simulink model "BasePerTracing_2023a"  (R2023a)
settings: Solver=FixedStepDiscrete  StartTime=0.0  StopTime=Inf  RelTol=1e-3  EnableMultiTasking=on
InitFcn:
  | mcb_pmsm_foc_qep_f28379d_data;
values from neighbouring files (symbols this model uses):
  ADCCount = ADCResolution-1    (= 4095)    [parameters.m]
  GainVsense = 4.99/(62+4.99)    (= 0.0744887296611)    [parameters.m]
  J = Jdc + Jbl    (= 7.32e-05)    [parameters.m]
  Km = 0.11    [parameters.m]
  Kpi = L/taui    (= 4.1)    [parameters.m]
  Kpv = J/(tauv*Km)    (= 0.0665454545455)    [parameters.m]
  OffsetADCINC4 = 2296    [parameters.m]
  PulseNumber = 2048*4    (= 8192)    [parameters.m]
  RadiantsPerCount = 2*pi/(PulseNumber-1)    (= 0.00076708403213)    [parameters.m]
  TaoFilterOffsetCurrent = 1    [parameters.m]
  TaoFilterOmega = 0.002    [parameters.m]
  Tii = L/R    (= 0.00128125)    [parameters.m]
  Tiv = Taom    (= 0.085)    [parameters.m]
  TSample = 0.0001    [parameters.m]
  VrefADC = 3    [parameters.m]
undefined symbols (not defined in the file or in its folder): dataType, Down, GPTRIP1SEL, GPTRIP2SEL, TZ1, TZ2, Up
libraries: c2802xlib x9, simulink x6, c280xlib x4, c2837xDlib x3, c2000lib x1, svdutilitieslib x1
(part 1 of 2)
settings Model: ExtModeTrigDuration=8  Creator=The MathWorks, Inc.  LastModifiedBy=student
settings SolverCC: AlgebraicLoopSolver=TrustRegion
settings OptimizationCC: DefaultParameterBehavior=Inlined  DefaultUnderspecifiedDataType=single  OptimizeBlockIOStorage=off  EnhancedBackFolding=on  InitFltsAndDblsToZero=on  NoFixptDivByZeroProtection=on  EfficientFloat2IntCast=on  EfficientMapNaN2IntZero=off  MaxStackSize=1024  OptimizeBlockOrder=speed  DifferentSizesBufferReuse=on  DenormalBehavior=FlushToZero  EfficientTunableParamExpr=on
settings DebuggingCC: MultiTaskDSMMsg=none  ParameterPrecisionLossMsg=none  ParameterTunabilityLossMsg=error  UnconnectedInputMsg=warning  UnconnectedOutputMsg=warning  UnconnectedLineMsg=warning
settings HardwareCC: ProdBitPerChar=16  ProdBitPerInt=16  ProdBitPerPointer=32  ProdBitPerSizeT=32  ProdBitPerPtrDiffT=32  ProdLargestAtomicInteger=Integer  ProdLargestAtomicFloat=None  ProdWordSize=16  ProdLongLongMode=on  ProdHWDeviceType=Texas Instruments->C2000
settings ModelReferenceCC: EnableRefExpFcnMdlSchedulingChecks=on
settings SFSimCC: MATLABDynamicMemAlloc=off
settings RTWCC: Description=Embedded Coder  SystemTargetFile=ert.tlc  HardwareBoard=TI Delfino F28379D LaunchPad  TemplateMakefile=ert_default_tmf  GenerateReport=on  Toolchain=Texas Instruments Code Composer Studio (C2000)  DLArmComputeVersion=19.05
settings CodeAppCC: IgnoreCustomStorageClasses=off  StateflowObjectComments=on
settings ERTTargetCC: CodeReplacementLibrary=TI C28x  ExtModeStaticAllocSize=10000  ConvertIfToSwitch=off  SuppressUnreachableDefaultCases=off  MemSecPackage=tic2000demospkg

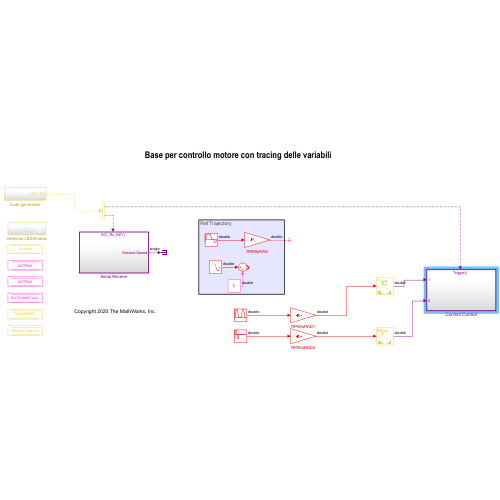
[thumbnail: Simulink's stored preview of the top-level diagram]
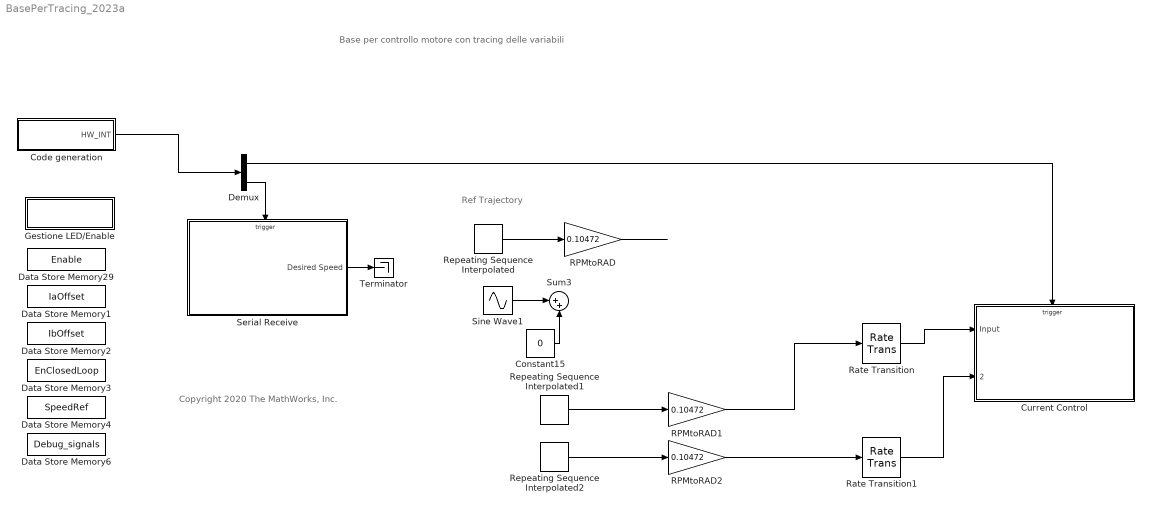
== system BasePerTracing_2023a ==
  note: Ref Trajectory
  note: Copyright 2020 The MathWorks, Inc.
  note: Base per controllo motore con tracing delle variabili
  Code generation : Subsystem
  Constant15 : Constant  Value=0
  Current Control : Subsystem
      settings: RTWSystemCode=Nonreusable function
  Data Store Memory1 : DataStoreMemory  DataStoreName=IaOffset  ReadBeforeWriteMsg=warning  WriteAfterWriteMsg=warning  WriteAfterReadMsg=warning  InitialValue=inverter.CtSensAOffset  ShowAdditionalParam=off
  Data Store Memory2 : DataStoreMemory  DataStoreName=IbOffset  ReadBeforeWriteMsg=warning  WriteAfterWriteMsg=warning  WriteAfterReadMsg=warning  InitialValue=inverter.CtSensBOffset  ShowAdditionalParam=off
  Data Store Memory29 : DataStoreMemory  DataStoreName=Enable  ReadBeforeWriteMsg=warning  WriteAfterWriteMsg=warning  WriteAfterReadMsg=warning  ShowAdditionalParam=off  OutDataTypeStr=boolean
  Data Store Memory3 : DataStoreMemory  DataStoreName=EnClosedLoop  ReadBeforeWriteMsg=warning  WriteAfterWriteMsg=warning  WriteAfterReadMsg=warning  ShowAdditionalParam=off  OutDataTypeStr=boolean
  Data Store Memory4 : DataStoreMemory  DataStoreName=SpeedRef  ShowAdditionalParam=off
  Data Store Memory6 : DataStoreMemory  DataStoreName=Debug_signals  ReadBeforeWriteMsg=warning  WriteAfterWriteMsg=warning  WriteAfterReadMsg=warning  InitialValue=5  ShowAdditionalParam=off  OutDataTypeStr=uint16
  Demux : Demux  Outputs=2
  Gestione LED/Enable : Subsystem
  RPMtoRAD : Gain  Gain=0.10472
  RPMtoRAD1 : Gain  Gain=0.10472
  RPMtoRAD2 : Gain  Gain=0.10472
  Rate Transition : RateTransition  Deterministic=off
  Rate Transition1 : RateTransition  Deterministic=off
  Repeating Sequence Interpolated : simulink/Sources/Repeating Sequence Interpolated  OutValues=[0 800 1000 1000 500 0 0 -500 -500 0].'  TimeValues=[0 0.3 0.5 1 1.2 1.4 1.7 2 2.2 2.5].'  LookUpMeth=Interpolation-Use End Values  tsamp=0.0001  OutMin=[]  OutMax=[]  OutDataTypeStr=double  OutputDataTypeScalingMode=double  OutDataType=fixdt(0,8)  OutScaling=2^-10
  Repeating Sequence Interpolated1 : simulink/Sources/Repeating Sequence Interpolated  OutValues="[0 700 700 0 0 710 710 0 0  ].'"  TimeValues=[0 0.055 0.1 0.15 0.25 0.305 0.35 0.40 0.45 ].'  LookUpMeth=Interpolation-Use End Values  tsamp=0.0001  OutMin=[]  OutMax=[]  OutDataTypeStr=double  OutputDataTypeScalingMode=double  OutDataType=fixdt(0,8)  OutScaling=2^-10
  Repeating Sequence Interpolated2 : simulink/Sources/Repeating Sequence Interpolated  OutValues=[0 12727 12727 0 0 -12727 -12727 0 0 0 0 0 0 ].'  TimeValues=[0 0.0001 0.055 0.0551 0.1 0.101 0.15 0.1501 0.25 0.305 0.35 0.40 0.45 ].'  LookUpMeth=Interpolation-Use End Values  tsamp=0.0001  OutMin=[]  OutMax=[]  OutDataTypeStr=double  OutputDataTypeScalingMode=double  OutDataType=fixdt(0,8)  OutScaling=2^-10
  Serial Receive : Subsystem  SystemSampleTime=1e-3
  Sine Wave1 : Sin  Amplitude=500  Frequency=15  SampleTime=0.0001
  Sum3 : Sum  Inputs=|++
  Terminator : Terminator
  wires:
  Code generation/1(HW_INT) -> Demux/1
  Demux/1 -> Current Control/Trigger
  Demux/2 -> Serial Receive/Trigger
  Serial Receive/1(Desired Speed) -> Terminator/1
  Rate Transition/1 -> Current Control/1(Input)
  Constant15/1 -> Sum3/2
  Repeating Sequence Interpolated/1 -> RPMtoRAD/1
  Sine Wave1/1 -> Sum3/1
  RPMtoRAD/1 -> ?
  Repeating Sequence Interpolated1/1 -> RPMtoRAD1/1
  RPMtoRAD1/1 -> Rate Transition/1
  Repeating Sequence Interpolated2/1 -> RPMtoRAD2/1
  RPMtoRAD2/1 -> Rate Transition1/1
  Rate Transition1/1 -> Current Control/2(2)

== system BasePerTracing_2023a/Code generation ==
  C28x Hardware Interrupt : c2000lib/Scheduling/C28x Hardware Interrupt  irqnumbers=[1 9]  pienumbers=[1 1]  irqpriorities=[30 50]  irqpreempts=[1 0]  showinput=off  dspchiptype=C280X
  HW_INT : Outport
  wires:
  C28x Hardware Interrupt/1 -> HW_INT/1

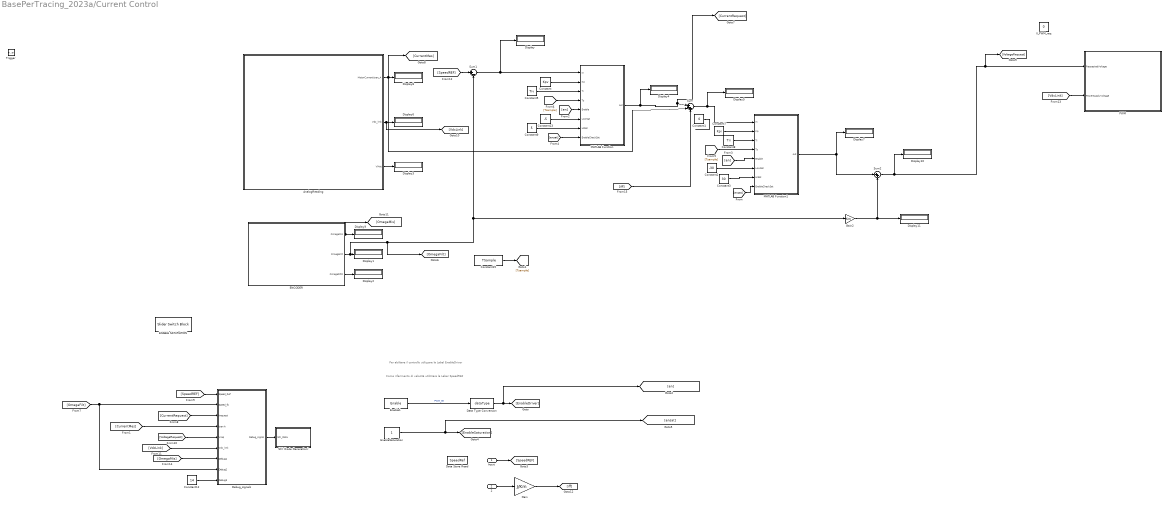
== system BasePerTracing_2023a/Current Control ==
  note: Per abilitare il controllo utilizzare la Label EnableDriver
  note: Come riferimento di velocità utilizzare la Laber SpeedREF
  Input : Inport
  2 : Inport  Port=2
  Trigger : TriggerPort  TriggerType=function-call  VariantControl=Variant  PortDimensions=1
  AnalogReading : Subsystem
  Constant : Constant  Value=Kpv
  Constant1 : Constant  Value=0
  Constant12 : Constant  Value=14
  Constant13 : Constant  Value=-5
  Constant15 : Constant  Value=TSample
  Constant2 : Constant  Value=-30
  Constant3 : Constant  Value=30
  Constant5 : Constant  Value=Tiv
  Constant7 : Constant  Value=Kpi
  Constant8 : Constant  Value=Tii
  Constant9 : Constant  Value=5
  Data Store Read : DataStoreRead  DataStoreName=SpeedRef  IndexOptions=Index vector (dialog)  Indices=1  OutputSizes=1
  Data Type Conversion : DataTypeConversion  OutDataTypeStr=dataType  SaturateOnIntegerOverflow=off  RndMeth=Floor
  Debug_signals : Subsystem
  Display{,1..11} (12 alike) : Display
  ENABLE SATURATION : SliderSwitchBlock
      settings: Values={{'Off', 'On'}, [0 1]}
  ENCODER : Subsystem
  Enable1 : DataStoreRead  DataStoreName=Enable  IndexOptions=Index vector (dialog)  Indices=1  OutputSizes=1
  EnableSaturation : Constant
  Gain : Gain  Gain=J/Km
  Gain2 : Gain  Gain=Km
  MATLAB Function : MATLAB Function  TreatAsAtomicUnit=on
  MATLAB Function1 : MATLAB Function  TreatAsAtomicUnit=on
  PWM : Subsystem
  SCI (Code Generation) : Subsystem
  Sum : Sum  Inputs=|+-+
  Sum1 : Sum  Inputs=|+-
  Sum2 : Sum  Inputs=|++
  V_PWM_req : Constant  Value=0
  wires:
  Debug_signals/1(Debug_signal) -> SCI (Code Generation)/1(SCI_Data)
  [CurrentMes] -> Debug_signals/4(Isen A)
  Enable1/1 -> Data Type Conversion/1  "PWM_En"
  [OmegaMis] -> Debug_signals/7(Debug1)
  [OmegaFilt] -> Debug_signals/2(Speed_fb), Debug_signals/8(Debug2)
  Constant12/1 -> Debug_signals/9(Debug3)
  [SpeedREF] -> Debug_signals/1(Speed_Ref)
  [VoltageRequest] -> Debug_signals/5(Vreq)
  [VdcLink] -> Debug_signals/6(Vdc_link)
  [CurrentRequest] -> Debug_signals/3(Irequest)
  MATLAB Function/1(out) -> Display4/1, [CurrentRequest], Sum/1
  [ensat] -> MATLAB Function1/8(EnableCheckSat)
  [en] -> MATLAB Function/5(Enable)
  Data Type Conversion/1 -> [en], [EnableDriver]
  [VdcLink] -> PWM/2(PowerSupplyVoltage)
  AnalogReading/1(MotorCurrent/Isen_A) -> [CurrentMes], Sum/2, Display8/1
  AnalogReading/3(VMot) -> Display3/1
  MATLAB Function1/1(out) -> Display7/1, Sum2/1
  Constant2/1 -> MATLAB Function1/6(LowSat)
  Constant9/1 -> MATLAB Function/7(HiSat)
  [Tsample] -> MATLAB Function1/4(Ts)
  Constant15/1 -> [Tsample]
  Sum2/1 -> [VoltageRequest], PWM/1(RequestedVoltage), Display10/1
  [ensat] -> MATLAB Function/8(EnableCheckSat)
  Constant5/1 -> MATLAB Function/3(Ti)
  AnalogReading/2(Vdc_link) -> [VdcLink], Display6/1
  [SpeedREF] -> Sum1/1
  EnableSaturation/1 -> [ensat], [EnableSaturation]
  Constant/1 -> MATLAB Function/2(Kp)
  Constant8/1 -> MATLAB Function1/3(Ti)
  Gain2/1 -> Sum2/2, Display11/1
  ENCODER/3(OmegaRPM) -> Display2/1
  [en] -> MATLAB Function1/5(Enable)
  ENCODER/2(OmegaFilt) -> [OmegaFilt], Sum1/2, Gain2/1, Display1/1
  Sum1/1 -> Display/1, MATLAB Function/1(in)
  Constant7/1 -> MATLAB Function1/2(Kp)
  Sum/1 -> MATLAB Function1/1(in), Display5/1
  Constant13/1 -> MATLAB Function/6(LowSat)
  Constant3/1 -> MATLAB Function1/7(HiSat)
  [Tsample] -> MATLAB Function/4(Ts)
  ENCODER/1(OmegaMis) -> [OmegaMis], Display9/1
  Input/1 -> [SpeedREF]
  2/1 -> Gain/1
  Gain/1 -> [iff]
  [iff] -> Sum/3
  Constant1/1 -> ?

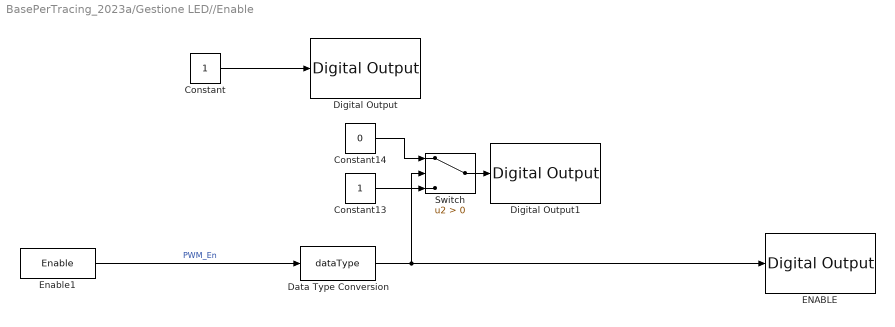
== system BasePerTracing_2023a/Gestione LED//Enable ==
  Constant : Constant  SampleTime=0.5
  Constant13 : Constant
  Constant14 : Constant  Value=0
  Data Type Conversion : DataTypeConversion  OutDataTypeStr=dataType  SaturateOnIntegerOverflow=off  RndMeth=Floor
  Digital Output : c2837xDlib/Digital Output  GPIO_Number=GPIO24~GPIO31  GPIO_Bit0=off  GPIO_BIT0_Toggle=off  GPIO_Bit1=off  GPIO_BIT1_Toggle=off  GPIO_Bit2=off  GPIO_BIT2_Toggle=off  GPIO_Bit3=off  GPIO_BIT3_Toggle=off  GPIO_Bit4=off  GPIO_BIT4_Toggle=off  GPIO_Bit5=off  GPIO_BIT5_Toggle=off  GPIO_Bit6=off  GPIO_BIT6_Toggle=off  GPIO_Bit7=on  GPIO_BIT7_Toggle=on
  Digital Output1 : c2837xDlib/Digital Output  GPIO_Number=GPIO32~GPIO39  GPIO_Bit0=off  GPIO_BIT0_Toggle=off  GPIO_Bit1=off  GPIO_BIT1_Toggle=off  GPIO_Bit2=on  GPIO_BIT2_Toggle=off  GPIO_Bit3=off  GPIO_BIT3_Toggle=off  GPIO_Bit4=off  GPIO_BIT4_Toggle=off  GPIO_Bit5=off  GPIO_BIT5_Toggle=off  GPIO_Bit6=off  GPIO_BIT6_Toggle=off  GPIO_Bit7=off  GPIO_BIT7_Toggle=off
  ENABLE : c2837xDlib/Digital Output  GPIO_Number=GPIO24~GPIO31  GPIO_Bit0=off  GPIO_BIT0_Toggle=off  GPIO_Bit1=off  GPIO_BIT1_Toggle=off  GPIO_Bit2=on  GPIO_BIT2_Toggle=off  GPIO_Bit3=off  GPIO_BIT3_Toggle=off  GPIO_Bit4=off  GPIO_BIT4_Toggle=off  GPIO_Bit5=off  GPIO_BIT5_Toggle=off  GPIO_Bit6=off  GPIO_BIT6_Toggle=off  GPIO_Bit7=off  GPIO_BIT7_Toggle=off
  Enable1 : DataStoreRead  DataStoreName=Enable  IndexOptions=Index vector (dialog)  Indices=1  OutputSizes=1
  Switch : Switch  Criteria=u2 > Threshold  SaturateOnIntegerOverflow=off  InputSameDT=off
  wires:
  Data Type Conversion/1 -> Switch/2, ENABLE/1
  Switch/1 -> Digital Output1/1
  Constant14/1 -> Switch/1
  Constant/1 -> Digital Output/1
  Enable1/1 -> Data Type Conversion/1  "PWM_En"
  Constant13/1 -> Switch/3

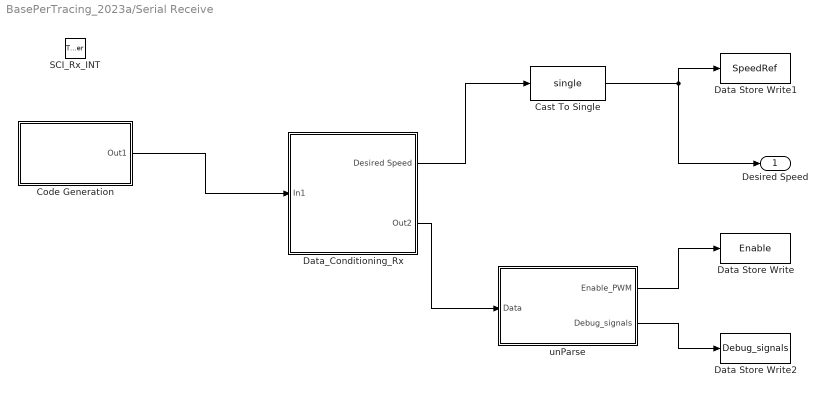
== system BasePerTracing_2023a/Serial Receive ==
  SCI_Rx_INT : TriggerPort  TriggerType=function-call  VariantControl=Variant
  Cast To Single : DataTypeConversion  OutDataTypeStr=single  SaturateOnIntegerOverflow=off  RndMeth=Floor
  Code Generation : Subsystem  Variant=on
  Data Store Write : DataStoreWrite  DataStoreName=Enable  IndexOptions=Index vector (dialog)  Indices=1  OutputSizes=1
  Data Store Write1 : DataStoreWrite  DataStoreName=SpeedRef  IndexOptions=Index vector (dialog)  Indices=1  OutputSizes=1
  Data Store Write2 : DataStoreWrite  DataStoreName=Debug_signals  IndexOptions=Index vector (dialog)  Indices=1  OutputSizes=1
  Data_Conditioning_Rx : Subsystem  Variant=on
  unParse : Subsystem
  Desired Speed : Outport  VectorParamsAs1DForOutWhenUnconnected=off
  wires:
  unParse/2(Debug_signals) -> Data Store Write2/1
  Data_Conditioning_Rx/2(Out2) -> unParse/1(Data)
  Code Generation/1(Out1) -> Data_Conditioning_Rx/1(In1)
  unParse/1(Enable_PWM) -> Data Store Write/1
  Data_Conditioning_Rx/1(Desired Speed) -> Cast To Single/1
  Cast To Single/1 -> Desired Speed/1, Data Store Write1/1

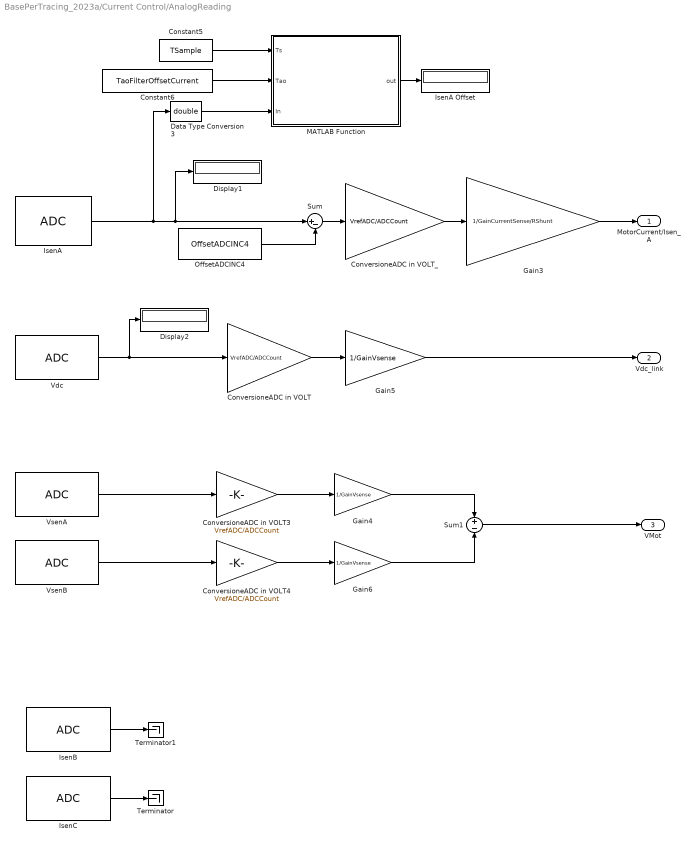
== system BasePerTracing_2023a/Current Control/AnalogReading ==
  Constant5 : Constant  Value=TSample  OutDataTypeStr=double
  Constant6 : Constant  Value=TaoFilterOffsetCurrent  OutDataTypeStr=double
  ConversioneADC in VOLT : Gain  Gain=VrefADC/ADCCount
  ConversioneADC in VOLT3 : Gain  Gain=VrefADC/ADCCount
  ConversioneADC in VOLT4 : Gain  Gain=VrefADC/ADCCount
  ConversioneADC in VOLT_ : Gain  Gain=VrefADC/ADCCount
  Data Type Conversion3 : DataTypeConversion  OutDataTypeStr=double  SaturateOnIntegerOverflow=off  RndMeth=Floor
  Display1 : Display
  Display2 : Display
  Gain3 : Gain  Gain=1/GainCurrentSense/RShunt
  Gain4 : Gain  Gain=1/GainVsense
  Gain5 : Gain  Gain=1/GainVsense
  Gain6 : Gain  Gain=1/GainVsense
  IsenA : c2802xlib/ADC  blkParamProc=C2000_Type4  ADCModule=C  samplingMode=Single sample mode  ADCResolution=12-bit (Single-ended input)  useSOC1=SOC0  useSOC2=SOC0_SOC1  SOCAcquisitionWindow=15  SOCTriggerSource=ePWM4_ADCSOCA  SOCInterruptTrigger=No ADCINT  Ts=-1  dType=uint16  postInterrupt=off  interruptSel=ADCINT1  ADCINTContinuous=on  endma=off  chdma=1  conv1=ADCINA0  conv2=ADCINA0 and ADCINB0  conv1_Type4=ADCIN4  conv2_Type4=ADCIN0 and ADCIN1
  IsenA Offset : Display
  IsenB : c2802xlib/ADC  blkParamProc=C2000_Type4  ADCModule=B  samplingMode=Single sample mode  ADCResolution=12-bit (Single-ended input)  useSOC1=SOC0  useSOC2=SOC0_SOC1  SOCAcquisitionWindow=15  SOCTriggerSource=ePWM4_ADCSOCA  SOCInterruptTrigger=No ADCINT  Ts=-1  dType=uint16  postInterrupt=off  interruptSel=ADCINT1  ADCINTContinuous=on  endma=off  chdma=1  conv1=ADCINA0  conv2=ADCINA0 and ADCINB0  conv1_Type4=ADCIN4  conv2_Type4=ADCIN0 and ADCIN1
  IsenC : c2802xlib/ADC  blkParamProc=C2000_Type4  ADCModule=A  samplingMode=Single sample mode  ADCResolution=12-bit (Single-ended input)  useSOC1=SOC0  useSOC2=SOC0_SOC1  SOCAcquisitionWindow=15  SOCTriggerSource=ePWM4_ADCSOCA  SOCInterruptTrigger=No ADCINT  Ts=-1  dType=uint16  postInterrupt=off  interruptSel=ADCINT1  ADCINTContinuous=on  endma=off  chdma=1  conv1=ADCINA0  conv2=ADCINA0 and ADCINB0  conv1_Type4=ADCIN4  conv2_Type4=ADCIN0 and ADCIN1
  MATLAB Function : MATLAB Function  TreatAsAtomicUnit=on
  OffsetADCINC4 : Constant  Value=OffsetADCINC4
  Sum : Sum  Inputs=|+-
  Sum1 : Sum  Inputs=+|-
  Terminator : Terminator
  Terminator1 : Terminator
  Vdc : c2802xlib/ADC  blkParamProc=C2000_Type4  ADCModule=A  samplingMode=Single sample mode  ADCResolution=12-bit (Single-ended input)  useSOC1=SOC1  useSOC2=SOC0_SOC1  SOCAcquisitionWindow=15  SOCTriggerSource=ePWM4_ADCSOCA  SOCInterruptTrigger=No ADCINT  Ts=-1  dType=uint16  postInterrupt=on  interruptSel=ADCINT1  ADCINTContinuous=on  endma=off  chdma=1  conv1=ADCINA0  conv2=ADCINA0 and ADCINB0  conv1_Type4=ADCIN5  conv2_Type4=ADCIN0 and ADCIN1
  VsenA : c2802xlib/ADC  blkParamProc=C2000_Type4  ADCModule=A  samplingMode=Single sample mode  ADCResolution=12-bit (Single-ended input)  useSOC1=SOC2  useSOC2=SOC0_SOC1  SOCAcquisitionWindow=15  SOCTriggerSource=ePWM4_ADCSOCA  SOCInterruptTrigger=No ADCINT  Ts=-1  dType=uint16  postInterrupt=on  interruptSel=ADCINT2  ADCINTContinuous=on  endma=off  chdma=1  conv1=ADCINA0  conv2=ADCINA0 and ADCINB0  conv1_Type4=ADCIN15  conv2_Type4=ADCIN0 and ADCIN1
  VsenB : c2802xlib/ADC  blkParamProc=C2000_Type4  ADCModule=C  samplingMode=Single sample mode  ADCResolution=12-bit (Single-ended input)  useSOC1=SOC3  useSOC2=SOC0_SOC1  SOCAcquisitionWindow=15  SOCTriggerSource=ePWM4_ADCSOCA  SOCInterruptTrigger=No ADCINT  Ts=-1  dType=uint16  postInterrupt=on  interruptSel=ADCINT3  ADCINTContinuous=on  endma=off  chdma=1  conv1=ADCINA0  conv2=ADCINA0 and ADCINB0  conv1_Type4=ADCIN5  conv2_Type4=ADCIN0 and ADCIN1
  MotorCurrent/Isen_A : Outport
  Vdc_link : Outport  Port=2
  VMot : Outport  Port=3
  wires:
  ConversioneADC in VOLT_/1 -> Gain3/1
  Data Type Conversion3/1 -> MATLAB Function/3(In)
  ConversioneADC in VOLT/1 -> Gain5/1
  Constant5/1 -> MATLAB Function/1(Ts)
  OffsetADCINC4/1 -> Sum/2
  IsenA/1 -> Data Type Conversion3/1, Sum/1, Display1/1
  Constant6/1 -> MATLAB Function/2(Tao)
  Sum/1 -> ConversioneADC in VOLT_/1
  MATLAB Function/1(out) -> IsenA Offset/1
  Vdc/1 -> Display2/1, ConversioneADC in VOLT/1
  Gain5/1 -> Vdc_link/1
  Gain3/1 -> MotorCurrent/Isen_A/1
  IsenC/1 -> Terminator/1
  IsenB/1 -> Terminator1/1
  Gain4/1 -> Sum1/1
  ConversioneADC in VOLT3/1 -> Gain4/1
  ConversioneADC in VOLT4/1 -> Gain6/1
  VsenB/1 -> ConversioneADC in VOLT4/1
  VsenA/1 -> ConversioneADC in VOLT3/1
  Sum1/1 -> VMot/1
  Gain6/1 -> Sum1/2

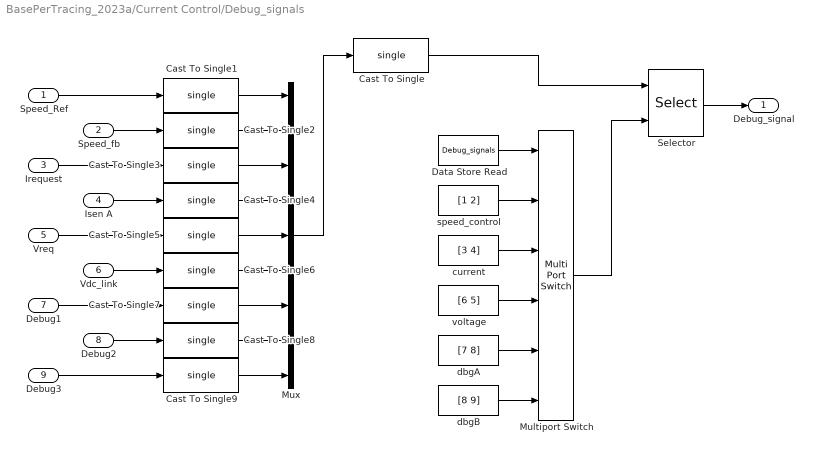
== system BasePerTracing_2023a/Current Control/Debug_signals ==
  Speed_Ref : Inport
  Speed_fb : Inport  Port=2
  Irequest : Inport  Port=3
  Isen A : Inport  Port=4
  Vreq : Inport  Port=5
  Vdc_link : Inport  Port=6
  Debug1 : Inport  Port=7
  Debug2 : Inport  Port=8
  Debug3 : Inport  Port=9
  Cast To Single{,1..9} (10 alike) : DataTypeConversion  OutDataTypeStr=single  SaturateOnIntegerOverflow=off  RndMeth=Floor
  Data Store Read : DataStoreRead  DataStoreName=Debug_signals  IndexOptions=Index vector (dialog)  Indices=1  OutputSizes=1
  Multiport Switch : MultiPortSwitch  Inputs=5  DiagnosticForDefault=Warning  OutDataTypeStr=uint16  RndMeth=Simplest  SaturateOnIntegerOverflow=off  InputSameDT=off
  Mux : Mux  Inputs=9
  Selector : Selector  InputPortWidth=9  IndexOptions=Index vector (port)  Indices=[1 3]  OutputSizes=1
  current : Constant  Value=[3 4]  OutDataTypeStr=uint16  SampleTime=-1
  dbgA : Constant  Value=[7 8]  OutDataTypeStr=uint16  SampleTime=-1
  dbgB : Constant  Value=[8 9]  OutDataTypeStr=uint16  SampleTime=-1
  speed_control : Constant  Value=[1 2]  OutDataTypeStr=uint16  SampleTime=-1
  voltage : Constant  Value=[6 5]  OutDataTypeStr=uint16  SampleTime=-1
  Debug_signal : Outport
  wires:
  speed_control/1 -> Multiport Switch/2
  current/1 -> Multiport Switch/3
  voltage/1 -> Multiport Switch/4
  dbgA/1 -> Multiport Switch/5
  dbgB/1 -> Multiport Switch/6
  Multiport Switch/1 -> Selector/2
  Data Store Read/1 -> Multiport Switch/1
  Selector/1 -> Debug_signal/1
  Irequest/1 -> Cast To Single3/1
  Isen A/1 -> Cast To Single4/1
  Speed_Ref/1 -> Cast To Single1/1
  Speed_fb/1 -> Cast To Single2/1
  Vreq/1 -> Cast To Single5/1
  Vdc_link/1 -> Cast To Single6/1
  Debug1/1 -> Cast To Single7/1
  Debug2/1 -> Cast To Single8/1
  Debug3/1 -> Cast To Single9/1
  Cast To Single/1 -> Selector/1
  Mux/1 -> Cast To Single/1
  Cast To Single1/1 -> Mux/1
  Cast To Single2/1 -> Mux/2
  Cast To Single3/1 -> Mux/3
  Cast To Single4/1 -> Mux/4
  Cast To Single5/1 -> Mux/5
  Cast To Single6/1 -> Mux/6
  Cast To Single7/1 -> Mux/7
  Cast To Single8/1 -> Mux/8
  Cast To Single9/1 -> Mux/9

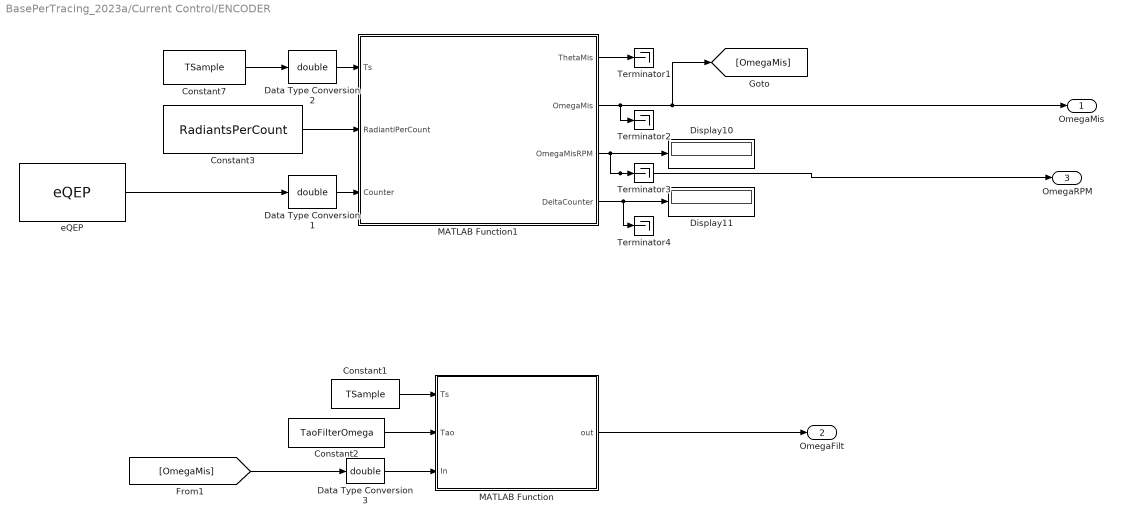
== system BasePerTracing_2023a/Current Control/ENCODER ==
  Constant1 : Constant  Value=TSample  OutDataTypeStr=double
  Constant2 : Constant  Value=TaoFilterOmega  OutDataTypeStr=double
  Constant3 : Constant  Value=RadiantsPerCount
  Constant7 : Constant  Value=TSample
  Data Type Conversion1 : DataTypeConversion  OutDataTypeStr=double  SaturateOnIntegerOverflow=off  RndMeth=Floor
  Data Type Conversion2 : DataTypeConversion  OutDataTypeStr=double  SaturateOnIntegerOverflow=off  RndMeth=Floor
  Data Type Conversion3 : DataTypeConversion  OutDataTypeStr=double  SaturateOnIntegerOverflow=off  RndMeth=Floor
  Display10 : Display
  Display11 : Display
  MATLAB Function : MATLAB Function  TreatAsAtomicUnit=on
  MATLAB Function1 : MATLAB Function  TreatAsAtomicUnit=on
  Terminator{1..4} (4 alike) : Terminator
  eQEP : c280xlib/eQEP  useModule=eQEP1  pcInputmode=Quadrature-count  externalClockrate=2x resolution: Count the rising/falling edge  swapPolarityselection=Counterclockwise  qdfOutputport=off  qapPolarityselection=off  qbpPolarityselection=off  qipPolarityselection=off  qspPolarityselection=off  igatePolarityselection=off  sampleTime=-1  pcOutputport=on  pcMaximumvalue=PulseNumber-1  indexInitializationcheck=off  indexInitializationevent=Rising edge  strobeInitializationcheck=off  strobeInitializationevent=Rising edge  softwareInitializationcheck=on  softwareInitializationsource=Set to init value at start up  softwareInitializationmode=on  pcInitialvalue=0  pcResetmode=Reset on the maximum position  ieloutputport=off  indexEventlatch=Rising edge  seloutputport=off  strobeEventlatch=Rising edge  pcefOutputport=off  enableEqepcapture=off  qctmrOutputport=off  qcprdOutputport=off  captureTimerprescaler=128  upEventprescaler=128  overflowErrorflag=off  directionErrorflag=off  captureTimerposition=On position counter read  unitTimerperiod=100000000  captureTimerlatch=off  capturePeriodlatch=off  positionCounterlatch=on  soenPolarityselection=off  spselPolarityselection=Index pin is used for sync output  compareValuesource=Specify via dialog  shadowMode=Load on QPOSCNT=0  compareValue=4294967295  syncOutputwidth=1  polaritySyncoutput=Active high  watchdogEnable=off  watchdogTimer=65535  outport1Datatype=auto  outport2Datatype=auto  outport3Datatype=auto  outport4Datatype=auto  outport5Datatype=auto  outport6Datatype=auto  outport7Datatype=auto  outport8Datatype=auto  outport9Datatype=auto  outport10Datatype=auto  outport11Datatype=auto  outport12Datatype=auto  eqepinterrupt_pce=off  eqepinterrupt_qpe=off  eqepinterrupt_qdc=off  eqepinterrupt_wto=off  eqepinterrupt_pcu=off  eqepinterrupt_pco=off  eqepinterrupt_pcr=off  eqepinterrupt_pcm=off  eqepinterrupt_sel=off  eqepinterrupt_iel=off  eqepinterrupt_uto=off  pheOutputport=off  watchdogOutputport=off  outport13Datatype=auto  outport14Datatype=auto
  OmegaMis : Outport
  OmegaFilt : Outport  Port=2
  OmegaRPM : Outport  Port=3
  wires:
  Constant3/1 -> MATLAB Function1/2(RadiantiPerCount)
  Constant7/1 -> Data Type Conversion2/1
  Data Type Conversion1/1 -> MATLAB Function1/3(Counter)
  eQEP/1 -> Data Type Conversion1/1
  MATLAB Function1/3(OmegaMisRPM) -> Display10/1, Terminator3/1, OmegaRPM/1
  MATLAB Function1/1(ThetaMis) -> Terminator1/1
  Data Type Conversion2/1 -> MATLAB Function1/1(Ts)
  MATLAB Function1/4(DeltaCounter) -> Terminator4/1, Display11/1
  MATLAB Function/1(out) -> OmegaFilt/1
  Constant1/1 -> MATLAB Function/1(Ts)
  Constant2/1 -> MATLAB Function/2(Tao)
  Data Type Conversion3/1 -> MATLAB Function/3(In)
  MATLAB Function1/2(OmegaMis) -> Terminator2/1, OmegaMis/1, [OmegaMis]
  [OmegaMis] -> Data Type Conversion3/1

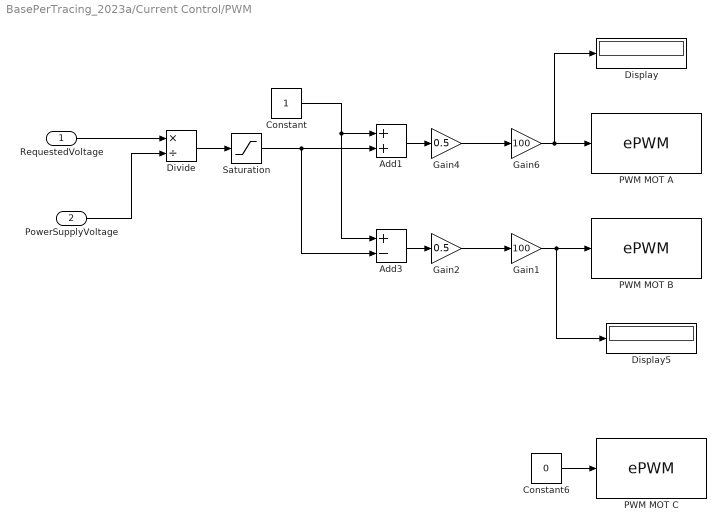
== system BasePerTracing_2023a/Current Control/PWM ==
  RequestedVoltage : Inport
  PowerSupplyVoltage : Inport  Port=2
  Add1 : Sum  AccumDataTypeStr=single
  Add3 : Sum  Inputs=+-  AccumDataTypeStr=single
  Constant : Constant
  Constant6 : Constant  Value=0
  Display : Display
  Display5 : Display
  Divide : Product  Inputs=*/  OutDataTypeStr=single
  Gain1 : Gain  Gain=100  OutDataTypeStr=single
  Gain2 : Gain  Gain=0.5  OutDataTypeStr=single
  Gain4 : Gain  Gain=0.5  OutDataTypeStr=single
  Gain6 : Gain  Gain=100  OutDataTypeStr=single
  PWM MOT A : c2802xlib/ePWM  PwmType=C2000_Type4  useModule=ePWM4  ePWMxLINKTBPRD=Not Linked  periodUnits=Clock cycles  timerSource=Specify via dialog  timerPeriod_clk=TBPRD  timerPeriod_sec=0.0001  tbshadow=Counter equals to zero  countingMode=Up-Down  phaseActiveEnable=Disable  phaseDirection=Count down after sync  phaseActive=0  synchronizationEnable=off  dcaevt1Sync=off  dcbevt1Sync=off  synchronizationOption=Counter equals to zero (CTR=Zero)  dcbevt1SyncOut=off  dcaevt1SyncOut=off  cmpdSyncOut=off  cmpcSyncOut=off  cmpbSyncOut=off  zeroSyncOut=on  swfSyncOut=off  perSynchronizationOption=Counter equals to period (CTR=PRD)  clockPrescale=1  HSclockPrescale=1  enswap=off  ePWMxAStatus=on  ePWMxAactionLogic1=Set  ePWMxAactionLogic2=Do nothing  ePWMxAactionLogic3=Clear  ePWMxAactionLogic4=Set  ePWMxAactionLogic5=Do nothing  ePWMxAactionLogic6=Do nothing  ePWMxACSFenable=off  ePWMxACSFvalue=Forcing disable  ePWMxASFreload=Zero  ePWMxBStatus=off  ePWMxBactionLogic1=Set  ePWMxBactionLogic2=Clear  ePWMxBactionLogic3=Do nothing  ePWMxBactionLogic4=Do nothing  ePWMxBactionLogic5=Clear  ePWMxBactionLogic6=Set  ePWMxBCSFenable=off  ePWMxBCSFvalue=Forcing disable  ePWMxBSFreload=Zero  ePWNxBOutWay=off  ePWMxLINKCMPA=Not Linked  CMPAUnits=Percentages  CMPASource=Input port  CMPAValue_per=0  CMPAValue_clk=2000  enCMPAshadow=Counter equals to zero (CTR=Zero)  ePWMxLINKCMPB=Not Linked  CMPBUnits=Clock cycles  CMPBSource=Specify via dialog  CMPBValue_per=50  CMPBValue_clk=2000  enCMPBshadow=Counter equals to zero (CTR=Zero)  ePWMxLINKCMPC=Not Linked  CMPCUnits=Clock cycles  CMPCSource=Specify via dialog  CMPCValue_per=50  CMPCValue_clk=32000  enCMPCshadow=Counter equals to zero (CTR=Zero)  ePWMxLINKCMPD=Not Linked  CMPDUnits=Clock cycles  CMPDSource=Specify via dialog  CMPDValue_per=50  CMPDValue_clk=32000  enCMPDshadow=Counter equals to zero (CTR=Zero)  enableDBePWMxA=on  enableDBePWMxB=on  enhalfcycle=off  DBpolarity=Active high complementary (AHC)  DBedgeDelay=Positive  DBSource_ePWMxA=ePWMxA  DBSource_ePWMxB=ePWMxA  DBPeriodUnits=Clock cycles  DBperiodSource=Specify via dialog  REDperiod=15  FEDperiod=15  REDperiod_sec=0  FEDperiod_sec=0  LoadModeDBRED=Immediate without using shadow  LoadModeDBFED=Immediate without using shadow  adcstartModuleA=on  adcrequestEventA=First event  adcstartEventA=Digital Compare Module A Event 1 start of conversion (DCAEVT1.soc)  adcstartEventA_type2=Counter equals to period (CTR=PRD)  adcstartModuleB=off  adcrequestEventB=First event  adcstartEventB=Counter equals to zero (CTR=Zero)  adcstartEventB_type2=Counter equals to zero (CTR=Zero)  intEn=off  intPrd=First event  intSel=Counter equals to zero (CTR=Zero)  intSel_type2=Counter equals to zero (CTR=Zero)  hrpe=off  enHRPWM=off  HRPWM_LoadMode=Counter equals to period (CTR=PRD)  HRPWM_CTLMode=Duty or Period control mode  HRPWM_EDGMode=Both edge  hrpeb=off  enHRPWMB=off  HRPWM_LoadModeB=Counter equals to zero (CTR=ZERO)  HRPWM_CTLModeB=Duty or Period control mode  HRPWM_EDGModeB=Both edge  enHRDBRED=off  enHRDBFED=off  enSFO=on  enautoconv=on  chopperEnable=off  chopperFrequency=1  chopperFirstwidth=1  chopperDuty=12.5%  tripZonesource=Specify via dialog  tzselOSHT1=off  tzselOSHT2=off  tzselOSHT3=off  tzselOSHDCAEV1=off  tzselOSHDCBEV1=off  tzselCBC1=off  tzselCBC2=off  tzselCBC3=off  tzselCBCDCAEV2=off  tzselCBCDCBEV2=off  tzselOSHT4=off  tzselOSHT5=off  tzselOSHT6=off  tzselCBC4=off  tzselCBC5=off  tzselCBC6=off  enTzOstIntr=off  enTzCbcIntr=off  enTzDCAEVT1Intr=off  enTzDCAEVT2Intr=off  enTzDCBEVT1Intr=off  enTzDCBEVT2Intr=off  ePWMxAforced=No action  ePWMxBforced=No action  DCAEVT1forced=No action  DCBEVT1forced=No action  DCAEVT2forced=No action  DCBEVT2forced=No action  dcah=Trip Zone 1 input (TZ1)  dcal=Trip Zone 2 input (TZ2)  dcbh=Trip Zone 1 input (TZ1)  dcbl=Trip Zone 2 input (TZ2)  dcah_type2=GPTRIP1SEL/(TZ1)  dcal_type2=GPTRIP2SEL/(TZ2)  dcbh_type2=GPTRIP1SEL/(TZ1)  dcbl_type2=GPTRIP2SEL/(TZ2)  gendcaevt1=Event disabled  gendcaevt2=Event disabled  gendcbevt1=Event disabled  gendcbevt2=Event disabled  dcaevt1src=DCAEVT1 with sync  dcaevt2src=DCAEVT2 with sync  dcbevt1src=DCBEVT1 with sync  dcbevt2src=DCBEVT2 with sync  pulsesel=Counter equals to zero (CTR=Zero)  blankinv=off  blankoffset=0  blankwidth=0  evsrcsel=Filtered version of DCAEVT1 (DCAEVT1FILT)  encape=off
  PWM MOT B : c2802xlib/ePWM  PwmType=C2000_Type4  useModule=ePWM5  ePWMxLINKTBPRD=Not Linked  periodUnits=Clock cycles  timerSource=Specify via dialog  timerPeriod_clk=TBPRD  timerPeriod_sec=0.0001  tbshadow=Counter equals to zero  countingMode=Up-Down  phaseActiveEnable=Set counter to phase value specified via dialog  phaseDirection=Count up after sync  phaseActive=0  synchronizationEnable=off  dcaevt1Sync=off  dcbevt1Sync=off  synchronizationOption=Pass through (EPWMxSYNCI or SWFSYNC)  dcbevt1SyncOut=off  dcaevt1SyncOut=off  cmpdSyncOut=off  cmpcSyncOut=off  cmpbSyncOut=off  zeroSyncOut=off  swfSyncOut=on  perSynchronizationOption=Counter equals to period (CTR=PRD)  clockPrescale=1  HSclockPrescale=1  enswap=off  ePWMxAStatus=on  ePWMxAactionLogic1=Set  ePWMxAactionLogic2=Do nothing  ePWMxAactionLogic3=Clear  ePWMxAactionLogic4=Set  ePWMxAactionLogic5=Do nothing  ePWMxAactionLogic6=Do nothing  ePWMxACSFenable=off  ePWMxACSFvalue=Forcing disable  ePWMxASFreload=Zero  ePWMxBStatus=off  ePWMxBactionLogic1=Set  ePWMxBactionLogic2=Clear  ePWMxBactionLogic3=Do nothing  ePWMxBactionLogic4=Do nothing  ePWMxBactionLogic5=Clear  ePWMxBactionLogic6=Set  ePWMxBCSFenable=off  ePWMxBCSFvalue=Forcing disable  ePWMxBSFreload=Zero  ePWNxBOutWay=off  ePWMxLINKCMPA=Not Linked  CMPAUnits=Percentages  CMPASource=Input port  CMPAValue_per=0  CMPAValue_clk=2000  enCMPAshadow=Counter equals to zero (CTR=Zero)  ePWMxLINKCMPB=Not Linked  CMPBUnits=Clock cycles  CMPBSource=Specify via dialog  CMPBValue_per=50  CMPBValue_clk=2000  enCMPBshadow=Counter equals to zero (CTR=Zero)  ePWMxLINKCMPC=Not Linked  CMPCUnits=Clock cycles  CMPCSource=Specify via dialog  CMPCValue_per=50  CMPCValue_clk=32000  enCMPCshadow=Counter equals to zero (CTR=Zero)  ePWMxLINKCMPD=Not Linked  CMPDUnits=Clock cycles  CMPDSource=Specify via dialog  CMPDValue_per=50  CMPDValue_clk=32000  enCMPDshadow=Counter equals to zero (CTR=Zero)  enableDBePWMxA=on  enableDBePWMxB=on  enhalfcycle=off  DBpolarity=Active high complementary (AHC)  DBedgeDelay=Positive  DBSource_ePWMxA=ePWMxA  DBSource_ePWMxB=ePWMxA  DBPeriodUnits=Clock cycles  DBperiodSource=Specify via dialog  REDperiod=15  FEDperiod=15  REDperiod_sec=0  FEDperiod_sec=0  LoadModeDBRED=Immediate without using shadow  LoadModeDBFED=Immediate without using shadow  adcstartModuleA=on  adcrequestEventA=First event  adcstartEventA=Digital Compare Module A Event 1 start of conversion (DCAEVT1.soc)  adcstartEventA_type2=Counter equals to zero (CTR=Zero)  adcstartModuleB=off  adcrequestEventB=First event  adcstartEventB=Counter equals to zero (CTR=Zero)  adcstartEventB_type2=Counter equals to zero (CTR=Zero)  intEn=off  intPrd=First event  intSel=Counter equals to zero (CTR=Zero)  intSel_type2=Counter equals to zero (CTR=Zero)  hrpe=off  enHRPWM=off  HRPWM_LoadMode=Counter equals to period (CTR=PRD)  HRPWM_CTLMode=Duty or Period control mode  HRPWM_EDGMode=Both edge  hrpeb=off  enHRPWMB=off  HRPWM_LoadModeB=Counter equals to zero (CTR=ZERO)  HRPWM_CTLModeB=Duty or Period control mode  HRPWM_EDGModeB=Both edge  enHRDBRED=off  enHRDBFED=off  enSFO=on  enautoconv=on  chopperEnable=off  chopperFrequency=1  chopperFirstwidth=1  chopperDuty=12.5%  tripZonesource=Specify via dialog  tzselOSHT1=off  tzselOSHT2=off  tzselOSHT3=off  tzselOSHDCAEV1=off  tzselOSHDCBEV1=off  tzselCBC1=off  tzselCBC2=off  tzselCBC3=off  tzselCBCDCAEV2=off  tzselCBCDCBEV2=off  tzselOSHT4=off  tzselOSHT5=off  tzselOSHT6=off  tzselCBC4=off  tzselCBC5=off  tzselCBC6=off  enTzOstIntr=off  enTzCbcIntr=off  enTzDCAEVT1Intr=off  enTzDCAEVT2Intr=off  enTzDCBEVT1Intr=off  enTzDCBEVT2Intr=off  ePWMxAforced=No action  ePWMxBforced=No action  DCAEVT1forced=No action  DCBEVT1forced=No action  DCAEVT2forced=No action  DCBEVT2forced=No action  dcah=Trip Zone 1 input (TZ1)  dcal=Trip Zone 2 input (TZ2)  dcbh=Trip Zone 1 input (TZ1)  dcbl=Trip Zone 2 input (TZ2)  dcah_type2=GPTRIP1SEL/(TZ1)  dcal_type2=GPTRIP2SEL/(TZ2)  dcbh_type2=GPTRIP1SEL/(TZ1)  dcbl_type2=GPTRIP2SEL/(TZ2)  gendcaevt1=Event disabled  gendcaevt2=Event disabled  gendcbevt1=Event disabled  gendcbevt2=Event disabled  dcaevt1src=DCAEVT1 with sync  dcaevt2src=DCAEVT2 with sync  dcbevt1src=DCBEVT1 with sync  dcbevt2src=DCBEVT2 with sync  pulsesel=Counter equals to zero (CTR=Zero)  blankinv=off  blankoffset=0  blankwidth=0  evsrcsel=Filtered version of DCAEVT1 (DCAEVT1FILT)  encape=off
  PWM MOT C : c2802xlib/ePWM  PwmType=C2000_Type4  useModule=ePWM6  ePWMxLINKTBPRD=Not Linked  periodUnits=Clock cycles  timerSource=Specify via dialog  timerPeriod_clk=TBPRD  timerPeriod_sec=0.0001  tbshadow=Counter equals to zero  countingMode=Up-Down  phaseActiveEnable=Set counter to phase value specified via dialog  phaseDirection=Count up after sync  phaseActive=0  synchronizationEnable=off  dcaevt1Sync=off  dcbevt1Sync=off  synchronizationOption=Pass through (EPWMxSYNCI or SWFSYNC)  dcbevt1SyncOut=off  dcaevt1SyncOut=off  cmpdSyncOut=off  cmpcSyncOut=off  cmpbSyncOut=off  zeroSyncOut=off  swfSyncOut=on  perSynchronizationOption=Counter equals to period (CTR=PRD)  clockPrescale=1  HSclockPrescale=1  enswap=off  ePWMxAStatus=on  ePWMxAactionLogic1=Set  ePWMxAactionLogic2=Do nothing  ePWMxAactionLogic3=Clear  ePWMxAactionLogic4=Set  ePWMxAactionLogic5=Do nothing  ePWMxAactionLogic6=Do nothing  ePWMxACSFenable=off  ePWMxACSFvalue=Forcing disable  ePWMxASFreload=Zero  ePWMxBStatus=off  ePWMxBactionLogic1=Set  ePWMxBactionLogic2=Clear  ePWMxBactionLogic3=Do nothing  ePWMxBactionLogic4=Do nothing  ePWMxBactionLogic5=Clear  ePWMxBactionLogic6=Set  ePWMxBCSFenable=off  ePWMxBCSFvalue=Forcing disable  ePWMxBSFreload=Zero  ePWNxBOutWay=off  ePWMxLINKCMPA=Not Linked  CMPAUnits=Percentages  CMPASource=Input port  CMPAValue_per=0  CMPAValue_clk=2000  enCMPAshadow=Counter equals to zero (CTR=Zero)  ePWMxLINKCMPB=Not Linked  CMPBUnits=Clock cycles  CMPBSource=Specify via dialog  CMPBValue_per=50  CMPBValue_clk=2000  enCMPBshadow=Counter equals to zero (CTR=Zero)  ePWMxLINKCMPC=Not Linked  CMPCUnits=Clock cycles  CMPCSource=Specify via dialog  CMPCValue_per=50  CMPCValue_clk=32000  enCMPCshadow=Counter equals to zero (CTR=Zero)  ePWMxLINKCMPD=Not Linked  CMPDUnits=Clock cycles  CMPDSource=Specify via dialog  CMPDValue_per=50  CMPDValue_clk=32000  enCMPDshadow=Counter equals to zero (CTR=Zero)  enableDBePWMxA=on  enableDBePWMxB=on  enhalfcycle=off  DBpolarity=Active high complementary (AHC)  DBedgeDelay=Positive  DBSource_ePWMxA=ePWMxA  DBSource_ePWMxB=ePWMxA  DBPeriodUnits=Clock cycles  DBperiodSource=Specify via dialog  REDperiod=15  FEDperiod=15  REDperiod_sec=0  FEDperiod_sec=0  LoadModeDBRED=Immediate without using shadow  LoadModeDBFED=Immediate without using shadow  adcstartModuleA=on  adcrequestEventA=First event  adcstartEventA=Digital Compare Module A Event 1 start of conversion (DCAEVT1.soc)  adcstartEventA_type2=Counter equals to zero (CTR=Zero)  adcstartModuleB=off  adcrequestEventB=First event  adcstartEventB=Counter equals to zero (CTR=Zero)  adcstartEventB_type2=Counter equals to zero (CTR=Zero)  intEn=off  intPrd=First event  intSel=Counter equals to zero (CTR=Zero)  intSel_type2=Counter equals to zero (CTR=Zero)  hrpe=off  enHRPWM=off  HRPWM_LoadMode=Counter equals to period (CTR=PRD)  HRPWM_CTLMode=Duty or Period control mode  HRPWM_EDGMode=Both edge  hrpeb=off  enHRPWMB=off  HRPWM_LoadModeB=Counter equals to zero (CTR=ZERO)  HRPWM_CTLModeB=Duty or Period control mode  HRPWM_EDGModeB=Both edge  enHRDBRED=off  enHRDBFED=off  enSFO=on  enautoconv=on  chopperEnable=off  chopperFrequency=1  chopperFirstwidth=1  chopperDuty=12.5%  tripZonesource=Specify via dialog  tzselOSHT1=off  tzselOSHT2=off  tzselOSHT3=off  tzselOSHDCAEV1=off  tzselOSHDCBEV1=off  tzselCBC1=off  tzselCBC2=off  tzselCBC3=off  tzselCBCDCAEV2=off  tzselCBCDCBEV2=off  tzselOSHT4=off  tzselOSHT5=off  tzselOSHT6=off  tzselCBC4=off  tzselCBC5=off  tzselCBC6=off  enTzOstIntr=off  enTzCbcIntr=off  enTzDCAEVT1Intr=off  enTzDCAEVT2Intr=off  enTzDCBEVT1Intr=off  enTzDCBEVT2Intr=off  ePWMxAforced=No action  ePWMxBforced=No action  DCAEVT1forced=No action  DCBEVT1forced=No action  DCAEVT2forced=No action  DCBEVT2forced=No action  dcah=Trip Zone 1 input (TZ1)  dcal=Trip Zone 2 input (TZ2)  dcbh=Trip Zone 1 input (TZ1)  dcbl=Trip Zone 2 input (TZ2)  dcah_type2=GPTRIP1SEL/(TZ1)  dcal_type2=GPTRIP2SEL/(TZ2)  dcbh_type2=GPTRIP1SEL/(TZ1)  dcbl_type2=GPTRIP2SEL/(TZ2)  gendcaevt1=Event disabled  gendcaevt2=Event disabled  gendcbevt1=Event disabled  gendcbevt2=Event disabled  dcaevt1src=DCAEVT1 with sync  dcaevt2src=DCAEVT2 with sync  dcbevt1src=DCBEVT1 with sync  dcbevt2src=DCBEVT2 with sync  pulsesel=Counter equals to zero (CTR=Zero)  blankinv=off  blankoffset=0  blankwidth=0  evsrcsel=Filtered version of DCAEVT1 (DCAEVT1FILT)  encape=off
  Saturation : Saturate  UpperLimit=0.95  LowerLimit=-0.95
  wires:
  Gain4/1 -> Gain6/1
  Constant/1 -> Add3/1, Add1/1
  Add3/1 -> Gain2/1
  Add1/1 -> Gain4/1
  Gain2/1 -> Gain1/1
  RequestedVoltage/1 -> Divide/1
  PowerSupplyVoltage/1 -> Divide/2
  Divide/1 -> Saturation/1
  Gain1/1 -> PWM MOT B/1, Display5/1
  Gain6/1 -> Display/1, PWM MOT A/1
  Constant6/1 -> PWM MOT C/1
  Saturation/1 -> Add3/2, Add1/2

== system BasePerTracing_2023a/Current Control/SCI (Code Generation) ==
  SCI_Data : Inport
  Data_Conditioning_Tx : Subsystem  Variant=on
  Data_Logging : Subsystem
  Demux2 : Demux  Outputs=2
  While Iterator Subsystem : Subsystem  TreatAsAtomicUnit=on
  wires:
  Demux2/2 -> While Iterator Subsystem/2(Iteration)  "SCI_Tx_Iteration"
  Demux2/1 -> While Iterator Subsystem/1(Data)  "SCI_Tx_Data"
  SCI_Data/1 -> Data_Conditioning_Tx/1(In1)
  Data_Logging/1(SCI_Tx) -> Demux2/1
  Data_Conditioning_Tx/1(Data_Log) -> Data_Logging/1(Data_Log)

== system BasePerTracing_2023a/Serial Receive/Code Generation ==
  Data_Type_Fixed_Point : Subsystem  VariantControl=~isequal(dataType, 'single')
  Data_Type_Float : Subsystem  VariantControl=isequal(dataType, 'single')
  Out1 : Outport

== system BasePerTracing_2023a/Serial Receive/Data_Conditioning_Rx ==
  In1 : Inport
  Data_Type_Fixed_Point : Subsystem  VariantControl=~isequal(dataType, 'single')
  Data_Type_Float : Subsystem  VariantControl=isequal(dataType, 'single')
  Desired Speed : Outport
  Out2 : Outport  Port=2

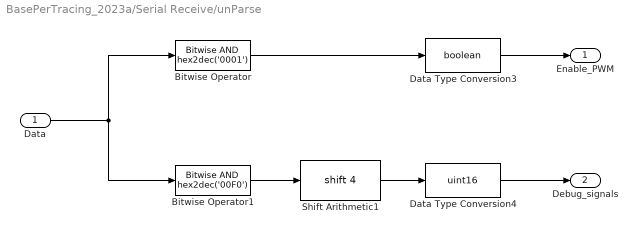
== system BasePerTracing_2023a/Serial Receive/unParse ==
  Data : Inport
  Bitwise Operator : simulink/Logic and Bit Operations/Bitwise Operator  logicop=AND  UseBitMask=on  BitMask=hex2dec('0001')  BitMaskRealWorld=Stored Integer
  Bitwise Operator1 : simulink/Logic and Bit Operations/Bitwise Operator  logicop=AND  UseBitMask=on  BitMask=hex2dec('00F0')  BitMaskRealWorld=Stored Integer
  Data Type Conversion3 : DataTypeConversion  OutDataTypeStr=boolean  RndMeth=Simplest  SaturateOnIntegerOverflow=off
  Data Type Conversion4 : DataTypeConversion  OutDataTypeStr=uint16  RndMeth=Simplest  SaturateOnIntegerOverflow=off
  Shift Arithmetic1 : ArithShift  BitShiftNumber=4
  Enable_PWM : Outport
  Debug_signals : Outport  Port=2
  wires:
  Bitwise Operator1/1 -> Shift Arithmetic1/1
  Data/1 -> Bitwise Operator/1, Bitwise Operator1/1
  Bitwise Operator/1 -> Data Type Conversion3/1
  Data Type Conversion4/1 -> Debug_signals/1
  Shift Arithmetic1/1 -> Data Type Conversion4/1
  Data Type Conversion3/1 -> Enable_PWM/1

== system BasePerTracing_2023a/Current Control/SCI (Code Generation)/Data_Conditioning_Tx ==
  In1 : Inport
  Data_Type_Fixed_Point : Subsystem  VariantControl=~isequal(dataType,'single')
  Data_Type_Float : Subsystem  VariantControl=isequal(dataType, 'single')
  Data_Log : Outport

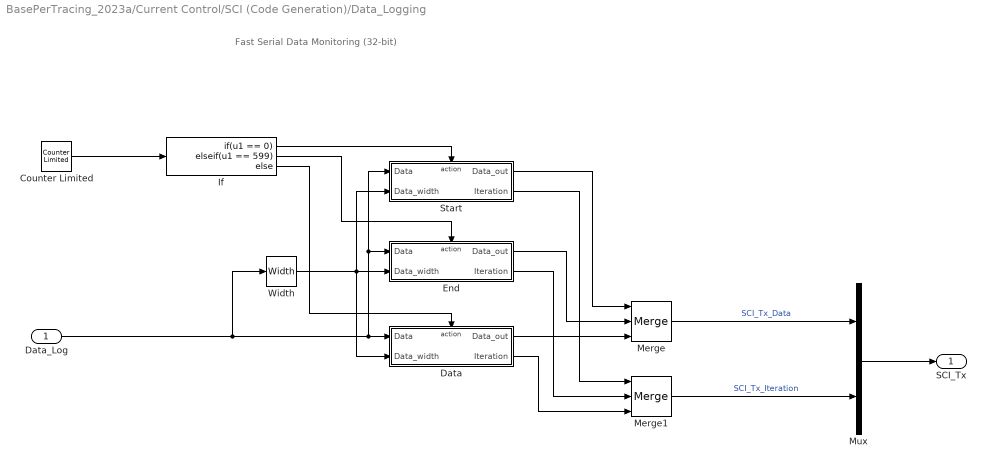
== system BasePerTracing_2023a/Current Control/SCI (Code Generation)/Data_Logging ==
  note: Fast Serial Data Monitoring (32-bit)
  Data_Log : Inport
  Counter Limited : simulink/Sources/Counter Limited  uplimit=600-1  tsamp=-1
  Data : Subsystem  TreatAsAtomicUnit=on
  End : Subsystem  TreatAsAtomicUnit=on
  If : If  IfExpression=u1 == 0  ElseIfExpressions=u1 == 599
  Merge : Merge  Inputs=3
  Merge1 : Merge  Inputs=3
  Mux : Mux  Inputs=2
  Start : Subsystem  TreatAsAtomicUnit=on
  Width : Width  OutDataTypeMode=All ports same datatype  DataType=uint16
  SCI_Tx : Outport
  wires:
  If/3 -> Data/Action
  Data/1(Data_out) -> Merge/3
  Width/1 -> Data/2(Data_width), Start/2(Data_width), End/2(Data_width)
  Merge/1 -> Mux/1  "SCI_Tx_Data"
  Counter Limited/1 -> If/1
  Start/2(Iteration) -> Merge1/1
  Start/1(Data_out) -> Merge/1
  If/2 -> End/Action
  Merge1/1 -> Mux/2  "SCI_Tx_Iteration"
  If/1 -> Start/Action
  End/1(Data_out) -> Merge/2
  End/2(Iteration) -> Merge1/2
  Data/2(Iteration) -> Merge1/3
  Mux/1 -> SCI_Tx/1
  Data_Log/1 -> Width/1, Start/1(Data), End/1(Data), Data/1(Data)

== system BasePerTracing_2023a/Current Control/SCI (Code Generation)/While Iterator Subsystem ==
  Data : Inport
  Iteration : Inport  Port=2
  Add : Sum  Inputs=+-  OutDataTypeStr=Inherit: Same as first input
  Index Vector : MultiPortSwitch  Inputs=1  SaturateOnIntegerOverflow=off  InputSameDT=off
  SCI Transmit : c280xlib/SCI Transmit  sciModule=A  dataHead=''  dataTail=''  frameSize=1  blockingMode=on  outputStatus=off
  While Iterator : WhileIterator  MaxIters=-1  WhileBlockType=do-while  ShowIterationPort=on  OutputDataType=int16
  wires:
  While Iterator/1 -> Add/2, Index Vector/1
  Data/1 -> Index Vector/2
  Index Vector/1 -> SCI Transmit/1
  Add/1 -> While Iterator/1
  Iteration/1 -> Add/1

== system BasePerTracing_2023a/Serial Receive/Code Generation/Data_Type_Fixed_Point ==
  SCI Receive : c280xlib/SCI Receive  sciModule=A  dataHead=''  headerCheckMaxCount=16  dataTail=''  dataType=uint32  dataLenOptions=Length via dialog  dataDim=2  maxDataLength=1  initValue=0  errOption=Output the last received value  errValue=0  sampleTime=-1  blockingMode=on  timeOut=0.00875  outputStatus=off
  Out1 : Outport
  wires:
  SCI Receive/1 -> Out1/1

== system BasePerTracing_2023a/Serial Receive/Code Generation/Data_Type_Float ==
  SCI Receive : c280xlib/SCI Receive  sciModule=A  dataHead=''  headerCheckMaxCount=16  dataTail=''  dataType=single  dataLenOptions=Length via dialog  dataDim=2  maxDataLength=1  initValue=0  errOption=Output the last received value  errValue=0  sampleTime=-1  blockingMode=on  timeOut=0.00875  outputStatus=off
  Out1 : Outport
  wires:
  SCI Receive/1 -> Out1/1

== system BasePerTracing_2023a/Serial Receive/Data_Conditioning_Rx/Data_Type_Fixed_Point ==
  In1 : Inport
  Data Type Conversion1 : DataTypeConversion  OutDataTypeStr=dataType  RndMeth=Simplest  SaturateOnIntegerOverflow=off
  Data Type Conversion2 : DataTypeConversion  OutDataTypeStr=fixdt(1,32,28)  ConvertRealWorld=Stored Integer (SI)  RndMeth=Simplest  SaturateOnIntegerOverflow=off
  Data Type Conversion3 : DataTypeConversion  OutDataTypeStr=uint16  RndMeth=Simplest  SaturateOnIntegerOverflow=off
  Demux : Demux  Outputs=2
  Desired Speed : Outport
  Out2 : Outport  Port=2
  wires:
  In1/1 -> Demux/1
  Data Type Conversion1/1 -> Desired Speed/1
  Data Type Conversion2/1 -> Data Type Conversion1/1
  Demux/1 -> Data Type Conversion2/1
  Demux/2 -> Data Type Conversion3/1
  Data Type Conversion3/1 -> Out2/1

== system BasePerTracing_2023a/Serial Receive/Data_Conditioning_Rx/Data_Type_Float ==
  In1 : Inport
  Data Type Conversion2 : DataTypeConversion  OutDataTypeStr=uint16  RndMeth=Simplest  SaturateOnIntegerOverflow=off
  Demux : Demux  Outputs=2
  Desired Speed : Outport
  Out2 : Outport  Port=2
  wires:
  In1/1 -> Demux/1
  Demux/1 -> Desired Speed/1
  Data Type Conversion2/1 -> Out2/1
  Demux/2 -> Data Type Conversion2/1

== system BasePerTracing_2023a/Current Control/SCI (Code Generation)/Data_Conditioning_Tx/Data_Type_Fixed_Point ==
  In1 : Inport
  Data Type Conversion : DataTypeConversion  OutDataTypeStr=fixdt(1,32,28)  RndMeth=Simplest  SaturateOnIntegerOverflow=off
  Data Type Conversion3 : DataTypeConversion  OutDataTypeStr=uint32  ConvertRealWorld=Stored Integer (SI)  RndMeth=Simplest  SaturateOnIntegerOverflow=off
  Data_Log : Outport
  wires:
  In1/1 -> Data Type Conversion/1
  Data Type Conversion3/1 -> Data_Log/1
  Data Type Conversion/1 -> Data Type Conversion3/1

== system BasePerTracing_2023a/Current Control/SCI (Code Generation)/Data_Conditioning_Tx/Data_Type_Float ==
  In1 : Inport
  Byte Pack : svdutilitieslib/Byte Pack  maskPackedDataType=uint32  datatypes={'single'}  byteAlign=4  blockPlatform=tic2000
  Data_Log : Outport
  wires:
  Byte Pack/1 -> Data_Log/1
  In1/1 -> Byte Pack/1

== system BasePerTracing_2023a/Current Control/SCI (Code Generation)/Data_Logging/Data ==
  Data : Inport
  Data_width : Inport  Port=2
  Action Port : ActionPort  ActionPortLabel=else
  Dummy : Constant  Value=hex2dec('0000')  OutDataTypeStr=uint32
  Mux : Mux  Inputs=2
  Data_out : Outport  VectorParamsAs1DForOutWhenUnconnected=off
  Iteration : Outport  Port=2  VectorParamsAs1DForOutWhenUnconnected=off
  wires:
  Data_width/1 -> Iteration/1
  Data/1 -> Mux/1
  Dummy/1 -> Mux/2
  Mux/1 -> Data_out/1

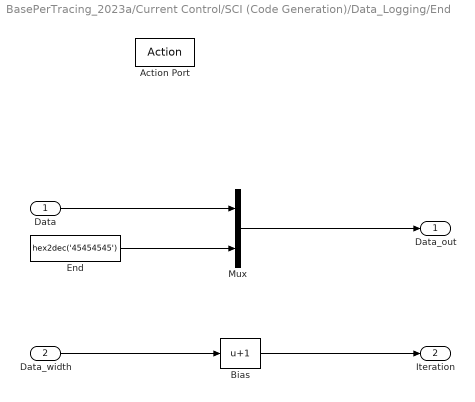
== system BasePerTracing_2023a/Current Control/SCI (Code Generation)/Data_Logging/End ==
  Data : Inport
  Data_width : Inport  Port=2
  Action Port : ActionPort  ActionPortLabel=elseif(u1 == 599)
  Bias : Bias  Bias=1  SaturateOnIntegerOverflow=off
  End : Constant  Value=hex2dec('45454545')  OutDataTypeStr=uint32
  Mux : Mux  Inputs=2
  Data_out : Outport  VectorParamsAs1DForOutWhenUnconnected=off
  Iteration : Outport  Port=2  VectorParamsAs1DForOutWhenUnconnected=off
  wires:
  Data/1 -> Mux/1
  Data_width/1 -> Bias/1
  Bias/1 -> Iteration/1
  End/1 -> Mux/2
  Mux/1 -> Data_out/1

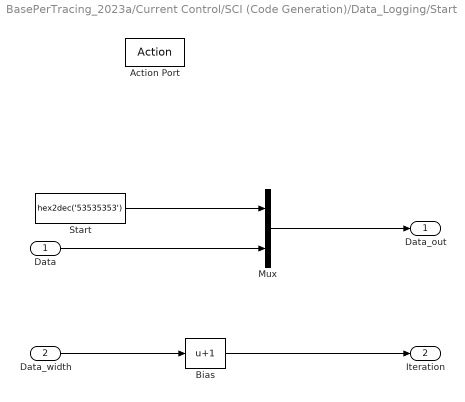
== system BasePerTracing_2023a/Current Control/SCI (Code Generation)/Data_Logging/Start ==
  Data : Inport
  Data_width : Inport  Port=2
  Action Port : ActionPort  ActionPortLabel=if(u1 == 0)
  Bias : Bias  Bias=1  SaturateOnIntegerOverflow=off
  Mux : Mux  Inputs=2
  Start : Constant  Value=hex2dec('53535353')  OutDataTypeStr=uint32
  Data_out : Outport  VectorParamsAs1DForOutWhenUnconnected=off
  Iteration : Outport  Port=2  VectorParamsAs1DForOutWhenUnconnected=off
  wires:
  Data/1 -> Mux/2
  Data_width/1 -> Bias/1
  Bias/1 -> Iteration/1
  Start/1 -> Mux/1
  Mux/1 -> Data_out/1

== matlab function BasePerTracing_2023a/Current Control/AnalogReading/MATLAB Function ==
  data: Ts input; out output; Tao input; In input
function out  = LowPassFilter(  Ts ,Tao, In)

persistent OutPrecedente
if isempty( OutPrecedente )
    OutPrecedente = 0 ;
end
    %Filtro passa basso discretizzato con il metodo delle differenze
    %all'indietro
    
    a=Ts/(Ts+Tao);
    b=Tao/(Ts+Tao);
    
    out=a*In+OutPrecedente*b;
   
    OutPrecedente = out;
   
end

== matlab function BasePerTracing_2023a/Current Control/ENCODER/MATLAB Function1 ==
  data: Ts input; ThetaMis output; RadiantiPerCount input; Counter input; OmegaMis output; OmegaMisRPM output; DeltaCounter output
function [ThetaMis, OmegaMis, OmegaMisRPM, DeltaCounter] = CounterToThetaOmega(Ts, RadiantiPerCount, Counter)

% Inizializzazione dei valori iniziali 
persistent CounterPrec  
if isempty( CounterPrec )
    CounterPrec = 0;
end 

    DeltaCounter=Counter-CounterPrec;
    
    if (DeltaCounter>double(0x1000))
        DeltaCounter=DeltaCounter-double(0x2000);
    end
    
    if (DeltaCounter<-double(0x1000))
        DeltaCounter=DeltaCounter+double(0x2000);
    end
        
    % conversione conteggio in radianti
    ThetaMis = Counter * RadiantiPerCount;
    
    DeltaThetaMis = DeltaCounter*RadiantiPerCount;
   
    OmegaMis = DeltaThetaMis/Ts;
    OmegaMisRPM=OmegaMis*60/(2*pi);
 
    CounterPrec= Counter;
end

== matlab function BasePerTracing_2023a/Current Control/MATLAB Function ==
  data: in input; out output; Kp input; Ti input; Ts input; Enable input; LowSat input; HiSat input; EnableCheckSat input
function out  = PI( in ,Kp , Ti , Ts , Enable, LowSat, HiSat, EnableCheckSat)
persistent in_prev out_prev
% Initial Value
if isempty( out_prev )
    out_prev = 0;
end
if isempty( in_prev )
    in_prev = 0;
end
% G(s)=(Kp/Ti)*((1+Ti*s)/s) (Tustin)
% We run control only if motor is running
if (Enable == 1)
    %I Calculate the output
    out = Kp*Ts/(2*Ti)*(in+in_prev) + Kp*(in-in_prev) + out_prev;
else
    out = 0;
    in = 0;
end  

if(EnableCheckSat == 1)
        %check for saturation
        if out > HiSat
            out = HiSat;
        elseif (out < LowSat)
            out = LowSat;
        end
end
    out_prev=out;
    in_prev=in;
end

== matlab function BasePerTracing_2023a/Current Control/MATLAB Function1 ==
  data: in input; out output; Kp input; Ti input; Ts input; Enable input; LowSat input; HiSat input; EnableCheckSat input
function out  = PI( in ,Kp , Ti , Ts , Enable, LowSat, HiSat, EnableCheckSat)
persistent in_prev out_prev
% Initial Value
if isempty( out_prev )
    out_prev = 0;
end
if isempty( in_prev )
    in_prev = 0;
end
% G(s)=(Kp/Ti)*((1+Ti*s)/s) (Tustin)
% We run control only if motor is running
if (Enable == 1)
    %I Calculate the output
    out = Kp*Ts/(2*Ti)*(in+in_prev) + Kp*(in-in_prev) + out_prev;
else
    out = 0;
    in = 0;
end
 if(EnableCheckSat == 1)
        %check for saturation
        if out > HiSat
            out = HiSat;
        elseif (out < LowSat)
            out = LowSat;
        end
 end
    out_prev=out;
    in_prev=in;
end
